simulink model "Automotive_Battery_Model"  (R2024b)
settings: Solver=VariableStepAuto  StartTime=0.0  StopTime=12  RelTol=1e-3
settings Model: Creator=Sajid  LastModifiedBy=Sajid

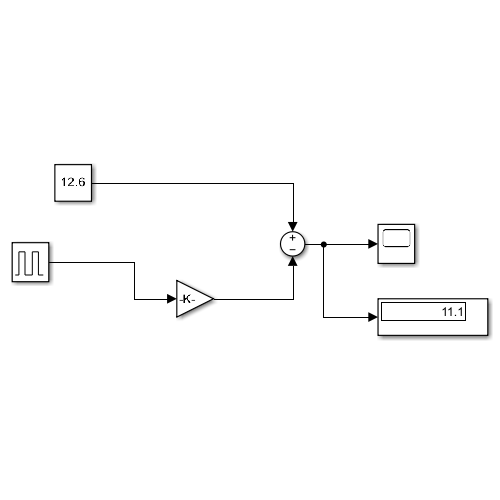
[thumbnail: Simulink's stored preview of the top-level diagram]
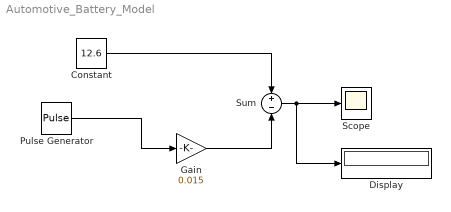
== system Automotive_Battery_Model ==
  Constant : Constant  Value=12.6
  Display : Display
  Gain : Gain  Gain=0.015
  Pulse Generator : DiscretePulseGenerator  PulseType=Time based  Amplitude=100  Period=5  PulseWidth=40  PhaseDelay=1
  Scope : Scope
  Sum : Sum  Inputs=+-
  wires:
  Pulse Generator/1 -> Gain/1
  Gain/1 -> Sum/2
  Constant/1 -> Sum/1
  Sum/1 -> Display/1, Scope/1
